simulink model "SimplifiedWTModelRL"  (R2018b)
settings: Solver=ode4  StartTime=0.0  StopTime=630  FixedStep=Parameter.Time.dt  RelTol=1e-3  EnableMultiTasking=on
values from neighbouring files (symbols this model uses):
  cP_modelrm = rmfield(cP_model,{'VarNames'})    [SimplifiedTurbine_Main.m]
  cT_modelrm = rmfield(cT_model,{'VarNames'})    [SimplifiedTurbine_Main.m]
  Parameter = SimplifiedTurbine_ParamterFile(Parameter)    [SimplifiedTurbine_Main.m]
libraries: simulink x3, S_TaLiRo x1
settings Model: Creator=212414199  LastModifiedBy=yoriyuki
settings DataIOCC: SaveFormat=Array
settings OptimizationCC: LifeSpan=inf
settings DebuggingCC: SolverPrmCheckMsg=warning  SFUnexpectedBacktrackingDiag=warning  SFNoUnconditionalDefaultTransitionDiag=warning  SFExecutionAtInitializationDiag=none
settings HardwareCC: ProdBitPerPointer=32  ProdBitPerSizeT=32  ProdBitPerPtrDiffT=32  ProdLargestAtomicFloat=None  ProdIntDivRoundTo=Undefined  ProdEndianess=Unspecified  ProdWordSize=32  ProdHWDeviceType=32-bit Generic
settings ModelReferenceCC: PropagateSignalLabelsOutOfModel=off
settings SFSimCC: SimUseLocalCustomCode=off
settings RTWCC: RTWUseLocalCustomCode=off
settings CodeAppCC: StateflowObjectComments=on
settings GRTTargetCC: TargetLangStandard=C89/C90 (ANSI)  GeneratePreprocessorConditionals=Disable all
settings ConfigComp: CovMetricSettings=dw  CovHtmlReporting=on  CovSaveCumulativeToWorkspaceVar=on  CovSaveSingleToWorkspaceVar=on  CovExternalEMLEnable=off  CovSFcnEnable=off

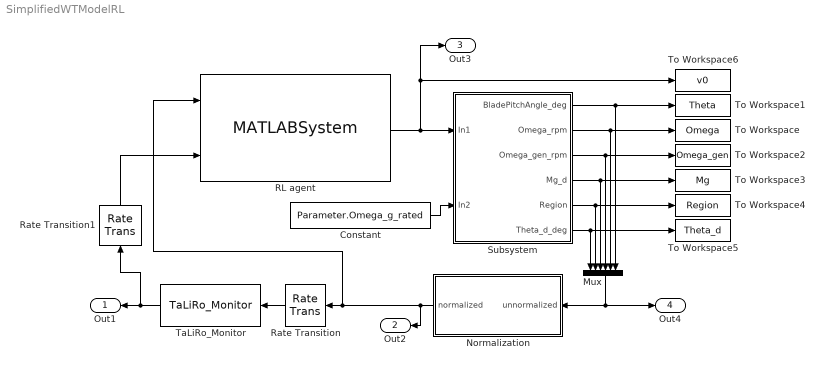
== system SimplifiedWTModelRL ==
  Constant : Constant  Value=Parameter.Omega_g_rated
  Mux : Mux  Inputs=6
  Normalization : MATLAB Function  TreatAsAtomicUnit=on
  RL agent : MATLABSystem  System=rl_agent_wind  sample_time=5  input_range=[8 16]  SimulateUsing=Code generation
      mask Type: rl_agent_wind
      mask Display:
      | disp('rl_agent_wind');
      | port_label('input',1,'state');
      | port_label('input',2,'reward');
      | port_label('output',1,'action');
  Rate Transition : RateTransition  OutPortSampleTime=0.1
  Rate Transition1 : RateTransition
  Subsystem : Subsystem
  TaLiRo_Monitor : S_TaLiRo/TaLiRo_Monitor  SFunctionModules=''
      settings: SourceProductName=S-TaLiRo
  To Workspace : ToWorkspace  VariableName=Omega  SaveFormat=Structure With Time  SampleTime=-1
  To Workspace1 : ToWorkspace  VariableName=Theta  SaveFormat=Structure With Time  SampleTime=-1
  To Workspace2 : ToWorkspace  VariableName=Omega_gen  SaveFormat=Structure With Time  SampleTime=-1
  To Workspace3 : ToWorkspace  VariableName=Mg  SaveFormat=Structure With Time  SampleTime=-1
  To Workspace4 : ToWorkspace  VariableName=Region  SaveFormat=Structure With Time  SampleTime=-1
  To Workspace5 : ToWorkspace  VariableName=Theta_d  SaveFormat=Structure With Time  SampleTime=-1
  To Workspace6 : ToWorkspace  VariableName=v0  SaveFormat=Structure With Time  SampleTime=-1
  Out1 : Outport
  Out2 : Outport  Port=2
  Out3 : Outport  Port=3
  Out4 : Outport  Port=4
  wires:
  RL agent/1 -> Subsystem/1(In1), Out3/1, To Workspace6/1
  Subsystem/1(BladePitchAngle_deg) -> Mux/6, To Workspace1/1
  Subsystem/2(Omega_rpm) -> Mux/5, To Workspace/1
  Subsystem/3(Omega_gen_rpm) -> Mux/4, To Workspace2/1
  Constant/1 -> Subsystem/2(In2)
  Subsystem/5(Region) -> Mux/2, To Workspace4/1
  Subsystem/6(Theta_d_deg) -> Mux/1, To Workspace5/1
  Subsystem/4(Mg_d) -> Mux/3, To Workspace3/1
  Mux/1 -> Out4/1, Normalization/1(unnormalized)
  TaLiRo_Monitor/1 -> Out1/1, Rate Transition1/1
  Normalization/1(normalized) -> Out2/1, RL agent/1, Rate Transition/1
  Rate Transition/1 -> TaLiRo_Monitor/1
  Rate Transition1/1 -> RL agent/2

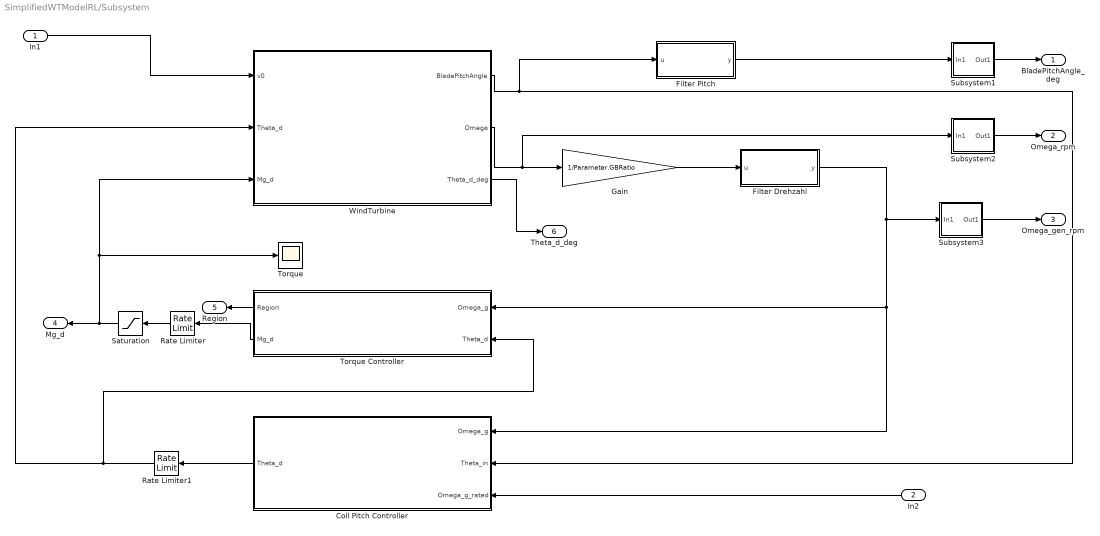
== system SimplifiedWTModelRL/Subsystem ==
  In1 : Inport
  In2 : Inport  Port=2
  Coll Pitch Controller : Subsystem
  Filter Drehzahl : Subsystem
  Filter Pitch : Subsystem
  Gain : Gain  Gain=1/Parameter.GBRatio
  Rate Limiter : RateLimiter  RisingSlewLimit=Parameter.VSControl.VS_MaxRat  FallingSlewLimit=-Parameter.VSControl.VS_MaxRat  SampleTimeMode=inherited
  Rate Limiter1 : RateLimiter  RisingSlewLimit=Parameter.Pitch.RateLimit  FallingSlewLimit=-Parameter.Pitch.RateLimit  SampleTimeMode=inherited  InitialCondition=Parameter.Pitch.ThetaDot0
  Saturation : Saturate  UpperLimit=Parameter.VSControl.VS_MaxTq  LowerLimit=-inf
  Subsystem1 : Subsystem
      mask Display: disp('rad2deg')
  Subsystem2 : Subsystem
      mask Display: disp('rad/s2rpm')
  Subsystem3 : Subsystem
      mask Display: disp('rad/s2rpm')
  Torque : Scope
  Torque Controller : MATLAB Function  TreatAsAtomicUnit=on
  WindTurbine : Subsystem
  BladePitchAngle_deg : Outport
  Omega_rpm : Outport  Port=2
  Omega_gen_rpm : Outport  Port=3
  Mg_d : Outport  Port=4
  Region : Outport  Port=5
  Theta_d_deg : Outport  Port=6
  wires:
  Subsystem1/1(Out1) -> BladePitchAngle_deg/1
  Torque Controller/2(Mg_d) -> Rate Limiter/1
  Subsystem3/1(Out1) -> Omega_gen_rpm/1
  Saturation/1 -> Mg_d/1, WindTurbine/3(Mg_d), Torque/1
  Rate Limiter/1 -> Saturation/1
  In1/1 -> WindTurbine/1(v0)
  WindTurbine/1(BladePitchAngle) -> Coll Pitch Controller/2(Theta_in), Filter Pitch/1(u)
  Filter Drehzahl/1(y) -> Torque Controller/1(Omega_g), Coll Pitch Controller/1(Omega_g), Subsystem3/1(In1)
  Subsystem2/1(Out1) -> Omega_rpm/1
  In2/1 -> Coll Pitch Controller/3(Omega_g_rated)
  Filter Pitch/1(y) -> Subsystem1/1(In1)
  Gain/1 -> Filter Drehzahl/1(u)
  Coll Pitch Controller/1(Theta_d) -> Rate Limiter1/1
  WindTurbine/2(Omega) -> Gain/1, Subsystem2/1(In1)
  Rate Limiter1/1 -> WindTurbine/2(Theta_d), Torque Controller/2(Theta_d)
  Torque Controller/1(Region) -> Region/1
  WindTurbine/3(Theta_d_deg) -> Theta_d_deg/1

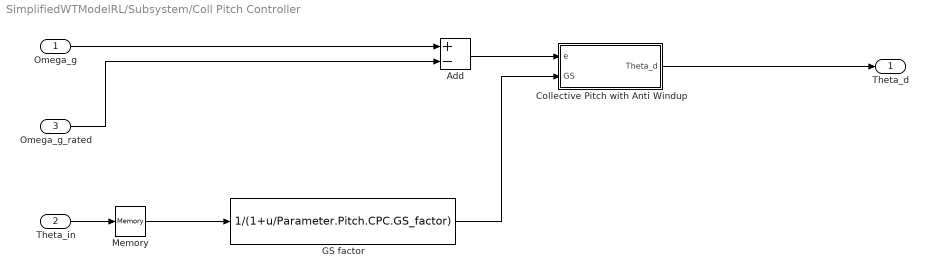
== system SimplifiedWTModelRL/Subsystem/Coll Pitch Controller ==
  Omega_g : Inport
  Theta_in : Inport  Port=2
  Omega_g_rated : Inport  Port=3
  Add : Sum  Inputs=+-
  Collective Pitch with Anti Windup : Subsystem
  "GS factor " : Fcn  Expr=1/(1+u/Parameter.Pitch.CPC.GS_factor)
  Memory : Memory  InitialCondition=Parameter.Pitch.Theta0
  Theta_d : Outport
  wires:
  Omega_g/1 -> Add/1
  Omega_g_rated/1 -> Add/2
  Theta_in/1 -> Memory/1
  Memory/1 -> "GS factor "/1
  Add/1 -> Collective Pitch with Anti Windup/1(e)
  "GS factor "/1 -> Collective Pitch with Anti Windup/2(GS)
  Collective Pitch with Anti Windup/1(Theta_d) -> Theta_d/1

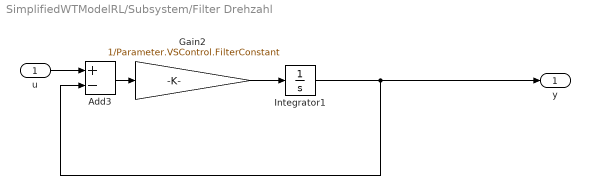
== system SimplifiedWTModelRL/Subsystem/Filter Drehzahl ==
  u : Inport
  Add3 : Sum  Inputs=+-
  Gain2 : Gain  Gain=1/Parameter.VSControl.FilterConstant  SaturateOnIntegerOverflow=on  OutDataTypeStr=Inherit: Same as input  ParamDataTypeStr=Inherit: Same as input
  Integrator1 : Integrator  InitialCondition=Parameter.Omega_g0
  y : Outport
  wires:
  Gain2/1 -> Integrator1/1
  Integrator1/1 -> Add3/2, y/1
  Add3/1 -> Gain2/1
  u/1 -> Add3/1

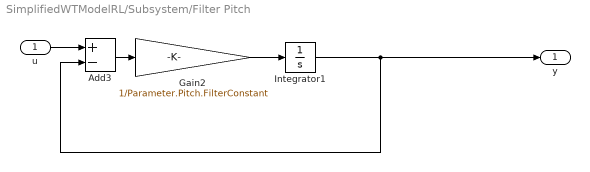
== system SimplifiedWTModelRL/Subsystem/Filter Pitch ==
  u : Inport
  Add3 : Sum  Inputs=+-
  Gain2 : Gain  Gain=1/Parameter.Pitch.FilterConstant  SaturateOnIntegerOverflow=on  OutDataTypeStr=Inherit: Same as input  ParamDataTypeStr=Inherit: Same as input
  Integrator1 : Integrator  InitialCondition=Parameter.Pitch.Theta0
  y : Outport
  wires:
  Gain2/1 -> Integrator1/1
  Integrator1/1 -> Add3/2, y/1
  Add3/1 -> Gain2/1
  u/1 -> Add3/1

== system SimplifiedWTModelRL/Subsystem/Subsystem1 ==
  In1 : Inport
  rad in deg : Gain  Gain=360/2/pi  SaturateOnIntegerOverflow=on  OutDataTypeStr=Inherit: Same as input  ParamDataTypeStr=Inherit: Same as input
  Out1 : Outport
  wires:
  In1/1 -> rad in deg/1
  rad in deg/1 -> Out1/1

== system SimplifiedWTModelRL/Subsystem/Subsystem2 ==
  In1 : Inport
  rad/s in rpm : Gain  Gain=60/2/pi  SaturateOnIntegerOverflow=on  OutDataTypeStr=Inherit: Same as input  ParamDataTypeStr=Inherit: Same as input
  Out1 : Outport
  wires:
  In1/1 -> rad/s in rpm/1
  rad/s in rpm/1 -> Out1/1

== system SimplifiedWTModelRL/Subsystem/Subsystem3 ==
  In1 : Inport
  rad/s in rpm : Gain  Gain=60/2/pi  SaturateOnIntegerOverflow=on  OutDataTypeStr=Inherit: Same as input  ParamDataTypeStr=Inherit: Same as input
  Out1 : Outport
  wires:
  In1/1 -> rad/s in rpm/1
  rad/s in rpm/1 -> Out1/1

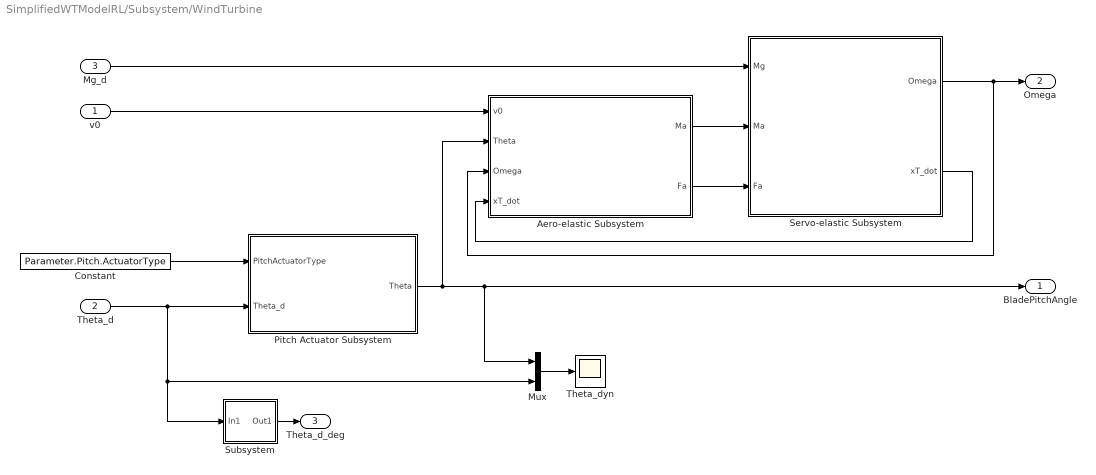
== system SimplifiedWTModelRL/Subsystem/WindTurbine ==
  v0 : Inport
  Theta_d : Inport  Port=2
  Mg_d : Inport  Port=3
  Aero-elastic Subsystem : Subsystem
  Constant : Constant  Value=Parameter.Pitch.ActuatorType
  Mux : Mux  Inputs=2
  Pitch Actuator Subsystem : Subsystem
  Servo-elastic Subsystem : Subsystem
  Subsystem : Subsystem
      mask Display: disp('rad2deg')
  "Theta_dyn " : Scope
  BladePitchAngle : Outport
  Omega : Outport  Port=2
  Theta_d_deg : Outport  Port=3
  wires:
  Constant/1 -> Pitch Actuator Subsystem/1("PitchActuatorType ")
  Theta_d/1 -> Mux/2, Subsystem/1(In1), Pitch Actuator Subsystem/2(Theta_d)
  Pitch Actuator Subsystem/1(Theta) -> Mux/1, BladePitchAngle/1, Aero-elastic Subsystem/2(Theta)
  Subsystem/1(Out1) -> Theta_d_deg/1
  v0/1 -> Aero-elastic Subsystem/1(v0)
  Aero-elastic Subsystem/1(Ma) -> Servo-elastic Subsystem/2(Ma)
  Aero-elastic Subsystem/2("Fa ") -> Servo-elastic Subsystem/3(Fa)
  Mg_d/1 -> Servo-elastic Subsystem/1(Mg)
  Servo-elastic Subsystem/1(Omega) -> Aero-elastic Subsystem/3(Omega), Omega/1
  Servo-elastic Subsystem/2("xT_dot ") -> Aero-elastic Subsystem/4(xT_dot)
  Mux/1 -> "Theta_dyn "/1

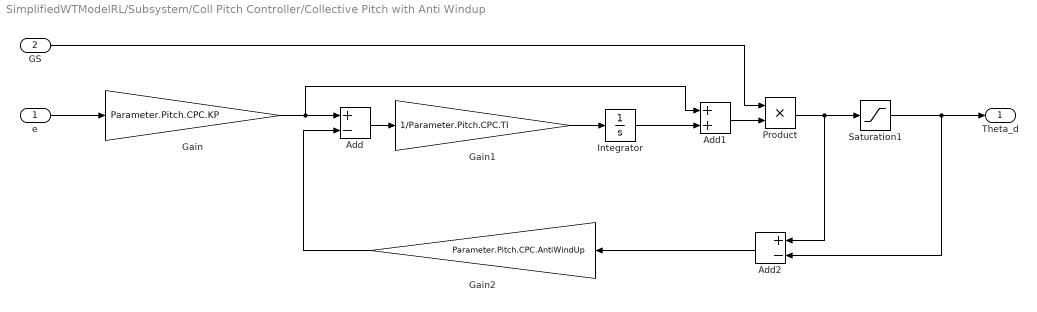
== system SimplifiedWTModelRL/Subsystem/Coll Pitch Controller/Collective Pitch with Anti Windup ==
  e : Inport
  GS : Inport  Port=2
  Add : Sum  Inputs=+-
  Add1 : Sum
  Add2 : Sum  Inputs=+-
  Gain : Gain  Gain=Parameter.Pitch.CPC.KP
  Gain1 : Gain  Gain=1/Parameter.Pitch.CPC.TI
  Gain2 : Gain  Gain=Parameter.Pitch.CPC.AntiWindUp
  Integrator : Integrator  InitialCondition=Parameter.Pitch.Theta0*(1+Parameter.Pitch.Theta0/Parameter.Pitch.CPC.GS_factor)
  Product : Product
  Saturation1 : Saturate  UpperLimit=Parameter.Pitch.Max  LowerLimit=Parameter.Pitch.Min
  Theta_d : Outport
  wires:
  e/1 -> Gain/1
  Gain/1 -> Add1/1, Add/1
  Add/1 -> Gain1/1
  Gain1/1 -> Integrator/1
  Add1/1 -> Product/2
  GS/1 -> Product/1
  Product/1 -> Add2/1, Saturation1/1
  Saturation1/1 -> Add2/2, Theta_d/1
  Add2/1 -> Gain2/1
  Gain2/1 -> Add/2
  Integrator/1 -> Add1/2

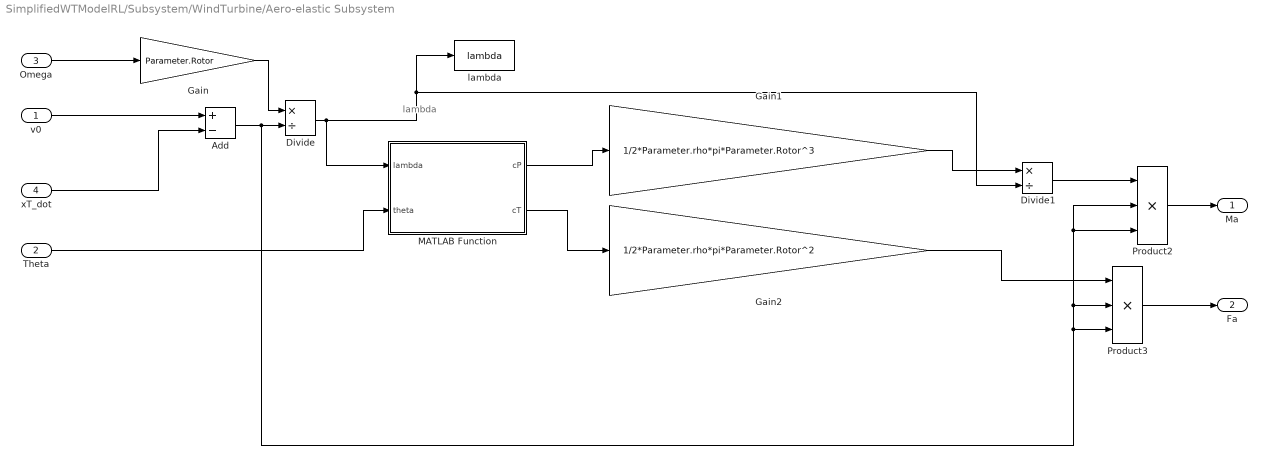
== system SimplifiedWTModelRL/Subsystem/WindTurbine/Aero-elastic Subsystem ==
  note: lambda
  v0 : Inport
  Theta : Inport  Port=2
  Omega : Inport  Port=3
  xT_dot : Inport  Port=4
  Add : Sum  Inputs=+-
  Divide : Product  Inputs=*/
  Divide1 : Product  Inputs=*/
  Gain : Gain  Gain=Parameter.Rotor
  Gain1 : Gain  Gain=1/2*Parameter.rho*pi*Parameter.Rotor^3
  Gain2 : Gain  Gain=1/2*Parameter.rho*pi*Parameter.Rotor^2
  MATLAB Function : MATLAB Function  TreatAsAtomicUnit=on
  Product2 : Product  Inputs=3  RndMeth=Zero
  Product3 : Product  Inputs=3  RndMeth=Zero
  "lambda " : ToWorkspace  VariableName=lambda  SaveFormat=Structure With Time  SampleTime=-1
  Ma : Outport
  "Fa " : Outport  Port=2
  wires:
  v0/1 -> Add/1
  xT_dot/1 -> Add/2
  Omega/1 -> Gain/1
  Gain/1 -> Divide/1
  Theta/1 -> MATLAB Function/2(theta)
  Divide/1 -> MATLAB Function/1(lambda), "lambda "/1, Divide1/2
  Gain1/1 -> Divide1/1
  Divide1/1 -> Product2/1
  Add/1 -> Divide/2, Product2/2, Product2/3, Product3/2, Product3/3
  Product2/1 -> Ma/1
  Gain2/1 -> Product3/1
  Product3/1 -> "Fa "/1
  MATLAB Function/1(cP) -> Gain1/1
  MATLAB Function/2(cT) -> Gain2/1

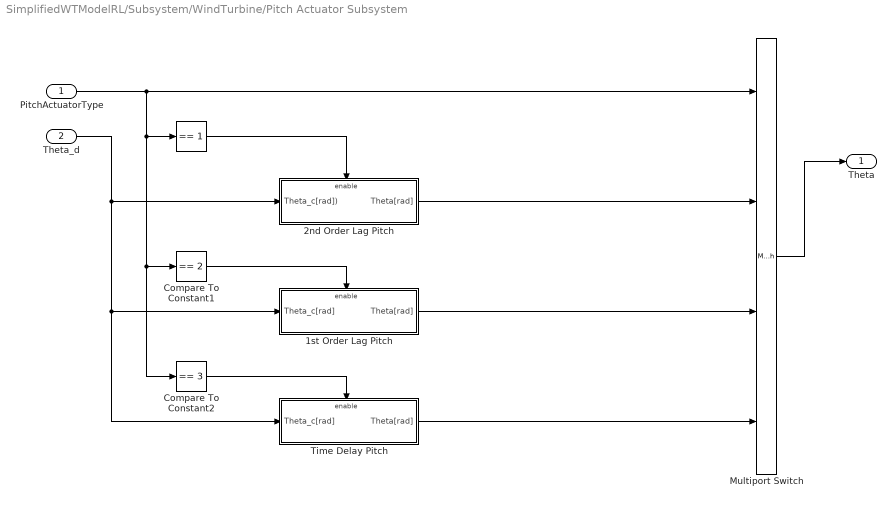
== system SimplifiedWTModelRL/Subsystem/WindTurbine/Pitch Actuator Subsystem ==
  "PitchActuatorType " : Inport
  Theta_d : Inport  Port=2
  " " : simulink/Logic and Bit Operations/Compare To Constant  relop===  const=1  OutDataTypeStr=boolean
  1st Order Lag Pitch : Subsystem  TreatAsAtomicUnit=on
  2nd Order Lag Pitch : Subsystem  TreatAsAtomicUnit=on
  Compare To Constant1 : simulink/Logic and Bit Operations/Compare To Constant  relop===  const=2  OutDataTypeStr=boolean
  Compare To Constant2 : simulink/Logic and Bit Operations/Compare To Constant  relop===  const=3  OutDataTypeStr=boolean
  Multiport Switch : MultiPortSwitch
  Time Delay Pitch : Subsystem  TreatAsAtomicUnit=on
  Theta : Outport
  wires:
  Multiport Switch/1 -> Theta/1
  Theta_d/1 -> Time Delay Pitch/1(Theta_c[rad]), 1st Order Lag Pitch/1(Theta_c[rad]), 2nd Order Lag Pitch/1(Theta_c[rad]))
  2nd Order Lag Pitch/1("Theta[rad] ") -> Multiport Switch/2
  1st Order Lag Pitch/1(Theta[rad]) -> Multiport Switch/3
  "PitchActuatorType "/1 -> " "/1, Compare To Constant1/1, Compare To Constant2/1, Multiport Switch/1
  Time Delay Pitch/1(Theta[rad]) -> Multiport Switch/4
  Compare To Constant1/1 -> 1st Order Lag Pitch/Enable
  " "/1 -> 2nd Order Lag Pitch/Enable
  Compare To Constant2/1 -> Time Delay Pitch/Enable

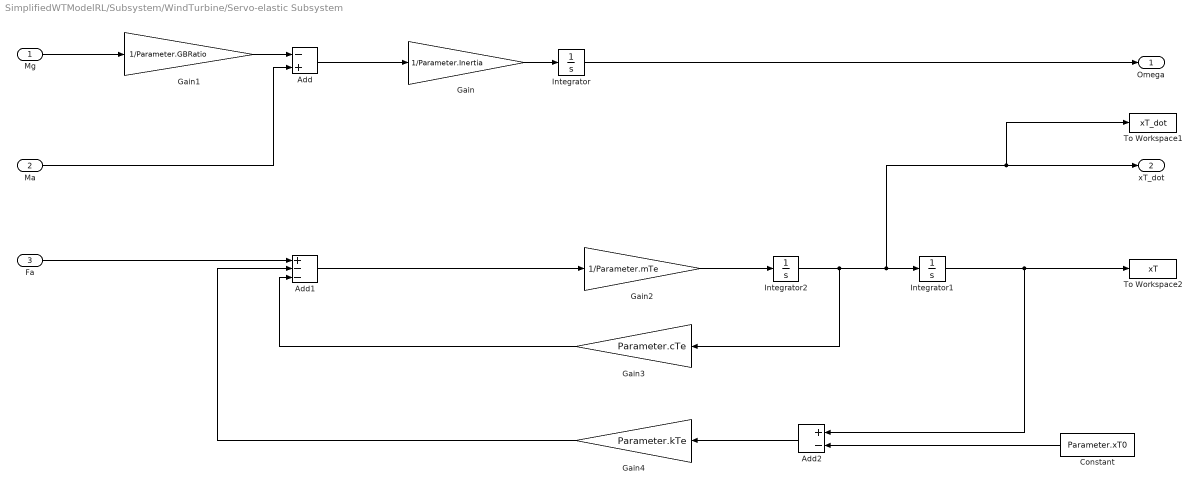
== system SimplifiedWTModelRL/Subsystem/WindTurbine/Servo-elastic Subsystem ==
  Mg : Inport
  Ma : Inport  Port=2
  Fa : Inport  Port=3
  Add : Sum  Inputs=-+
  Add1 : Sum  Inputs=+--
  Add2 : Sum  Inputs=+-
  Constant : Constant  Value=Parameter.xT0
  Gain : Gain  Gain=1/Parameter.Inertia
  Gain1 : Gain  Gain=1/Parameter.GBRatio
  Gain2 : Gain  Gain=1/Parameter.mTe
  Gain3 : Gain  Gain=Parameter.cTe
  Gain4 : Gain  Gain=Parameter.kTe
  Integrator : Integrator  InitialCondition=Parameter.Omega0
  Integrator1 : Integrator  InitialCondition=Parameter.xT0
  Integrator2 : Integrator  InitialCondition=Parameter.xt_dot0
  To Workspace1 : ToWorkspace  VariableName=xT_dot  SaveFormat=Structure With Time  SampleTime=-1
  To Workspace2 : ToWorkspace  VariableName=xT  SaveFormat=Structure With Time  SampleTime=-1
  Omega : Outport
  "xT_dot " : Outport  Port=2
  wires:
  Integrator/1 -> Omega/1
  Gain/1 -> Integrator/1
  Mg/1 -> Gain1/1
  Gain1/1 -> Add/1
  Ma/1 -> Add/2
  Add/1 -> Gain/1
  Integrator1/1 -> To Workspace2/1, Add2/1
  Integrator2/1 -> To Workspace1/1, "xT_dot "/1, Integrator1/1, Gain3/1
  Gain2/1 -> Integrator2/1
  Fa/1 -> Add1/1
  Add1/1 -> Gain2/1
  Gain3/1 -> Add1/3
  Gain4/1 -> Add1/2
  Add2/1 -> Gain4/1
  Constant/1 -> Add2/2

== system SimplifiedWTModelRL/Subsystem/WindTurbine/Subsystem ==
  In1 : Inport
  rad in deg : Gain  Gain=360/2/pi  SaturateOnIntegerOverflow=on  OutDataTypeStr=Inherit: Same as input  ParamDataTypeStr=Inherit: Same as input
  Out1 : Outport
  wires:
  In1/1 -> rad in deg/1
  rad in deg/1 -> Out1/1

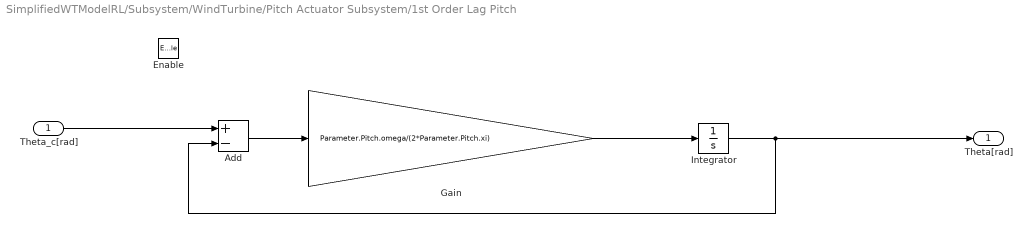
== system SimplifiedWTModelRL/Subsystem/WindTurbine/Pitch Actuator Subsystem/1st Order Lag Pitch ==
  Theta_c[rad] : Inport
  Enable : EnablePort
  Add : Sum  Inputs=+-
  Gain : Gain  Gain=Parameter.Pitch.omega/(2*Parameter.Pitch.xi)
  Integrator : Integrator  InitialCondition=Parameter.Pitch.Theta0
  Theta[rad] : Outport
  wires:
  Theta_c[rad]/1 -> Add/1
  Add/1 -> Gain/1
  Gain/1 -> Integrator/1
  Integrator/1 -> Theta[rad]/1, Add/2

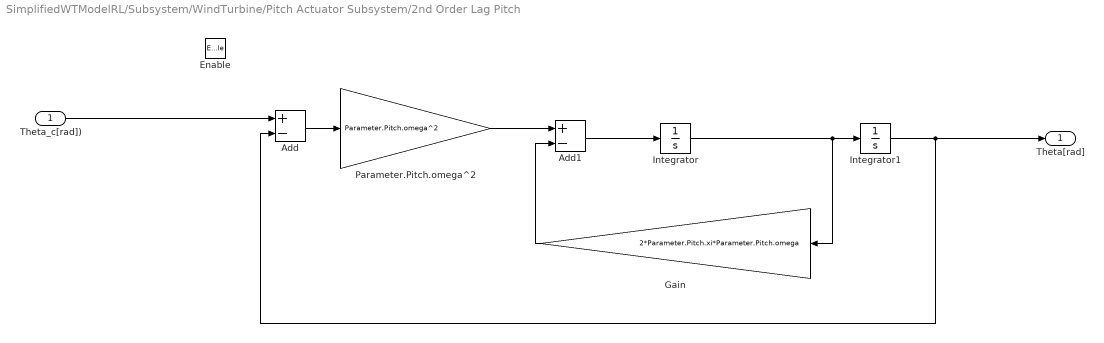
== system SimplifiedWTModelRL/Subsystem/WindTurbine/Pitch Actuator Subsystem/2nd Order Lag Pitch ==
  Theta_c[rad]) : Inport
  Enable : EnablePort
  Add : Sum  Inputs=+-
  Add1 : Sum  Inputs=+-
  Gain : Gain  Gain=2*Parameter.Pitch.xi*Parameter.Pitch.omega
  Integrator : Integrator  InitialCondition=Parameter.Pitch.ThetaDot0
  Integrator1 : Integrator  InitialCondition=Parameter.Pitch.Theta0
  Parameter.Pitch.omega^2 : Gain  Gain=Parameter.Pitch.omega^2
  "Theta[rad] " : Outport
  wires:
  Theta_c[rad])/1 -> Add/1
  Integrator1/1 -> "Theta[rad] "/1, Add/2
  Add/1 -> Parameter.Pitch.omega^2/1
  Parameter.Pitch.omega^2/1 -> Add1/1
  Gain/1 -> Add1/2
  Add1/1 -> Integrator/1
  Integrator/1 -> Gain/1, Integrator1/1

== system SimplifiedWTModelRL/Subsystem/WindTurbine/Pitch Actuator Subsystem/Time Delay Pitch ==
  Theta_c[rad] : Inport
  Enable : EnablePort
  Transport Delay : TransportDelay  DelayTime=Parameter.Pitch.Delay  InitialOutput=Parameter.Pitch.Theta0
  Theta[rad] : Outport
  wires:
  Theta_c[rad]/1 -> Transport Delay/1
  Transport Delay/1 -> Theta[rad]/1

== matlab function SimplifiedWTModelRL/Subsystem/WindTurbine/Aero-elastic Subsystem/MATLAB Function ==
  data: lambda input; cP output; theta input; cP_modelrm parameter; cT output; cT_modelrm parameter
function [cP,cT] = AeromapsPoly(lambda,theta,cP_modelrm, cT_modelrm)
%#eml

eml.extrinsic('polyvaln');

cP = 0.482;
cT = 0;


cP = polyvaln(cP_modelrm,[lambda,theta]);
cT = polyvaln(cT_modelrm,[lambda,theta]);

== matlab function SimplifiedWTModelRL/Subsystem/Torque Controller ==
  data: Region output; Omega_g input; Theta_d input; Mg_d output; Parameter parameter
function [Region, Mg_d] = VSTorqueController(Omega_g,Theta_d,Parameter)

% Code taken from NREL 5MW WT controller file (DISCON.f90)
VS_RtGnSp  = Parameter.VSControl.VS_RtGnSp;
VS_Rgn2K   = Parameter.VSControl.VS_Rgn2K;
VS_Rgn2Sp  = Parameter.VSControl.VS_Rgn2Sp;
VS_CtInSp  = Parameter.VSControl.VS_CtInSp;
VS_RtPwr   = Parameter.VSControl.VS_RtPwr;
VS_Rgn3MP  = Parameter.VSControl.VS_Rgn3MP;

VS_SySp    = Parameter.VSControl.VS_SySp;
VS_Slope15 = Parameter.VSControl.VS_Slope15;
VS_Slope25 = Parameter.VSControl.VS_Slope25;
VS_TrGnSp  = Parameter.VSControl.VS_TrGnSp;

GenSpeedF  = Omega_g;
PitCom     = Theta_d;

%Initialization
%Mg_d =VS_Rgn2K.*VS_RtGnSp.*VS_RtGnSp;

% Compute the generator torque, which depends on which region we are in:
if ((GenSpeedF >= VS_RtGnSp) || (PitCom >= VS_Rgn3MP)) % We are in region 3 - power is constant
    GenTrq = VS_RtPwr./GenSpeedF;
    Region = 3;
elseif (GenSpeedF <= VS_CtInSp)                                   % We are in region 1 - torque is zero
    GenTrq = 0.0;
    Region = 1;
elseif (GenSpeedF < VS_Rgn2Sp)                                    % We are in region 1 1/2 - linear ramp in torque from zero to optimal
    GenTrq = VS_Slope15.*(GenSpeedF - VS_CtInSp);
    Region = 1.5;
elseif (GenSpeedF <  VS_TrGnSp)                                   % We are in region 2 - optimal torque is proportional to the square of the generator speed
    GenTrq = VS_Rgn2K.*GenSpeedF.*GenSpeedF;
    Region = 2;
else                                                              % We are in region 2 1/2 - simple induction generator transition region
    GenTrq = VS_Slope25*(GenSpeedF - VS_SySp);
    Region = 2.5;
end

Mg_d = GenTrq;

%% This is done in Simulink, not here!!
% % Saturate the commanded torque using the maximum torque limit:
% 
% GenTrq  = min(GenTrq,VS_MaxTq);   % Saturate the command using the maximum torque limit
% 
% 
% % Saturate the commanded torque using the torque rate limit:
% % Initialize the value of LastGenTrq on the first pass only
% TrqRate = (GenTrq - LastGenTrq )/ElapTime;              % Torque rate (unsaturated)
% TrqRate = min(max(TrqRate, -VS_MaxRat ),VS_MaxRat);   % Saturate the torque rate using its maximum absolute value
% GenTrq  = LastGenTrq + TrqRate*ElapTime                  % Saturate the command using the torque rate limit

== matlab function SimplifiedWTModelRL/Normalization ==
  data: unnormalized input; normalized output
function normalized = normalize(unnormalized)
output_range = [0.0 13.0; 1.0 3.0; 2.50*10^4 5.0*10^4; 1000.0 1300.0; 10.0 13.0;0.0 13.0];
lower = output_range(:,1);
upper = output_range(:,2);
middle = (lower + upper)/2;
d = (upper - lower)/2;
normalized = (unnormalized - middle) ./ d;
